simulink model "ASM_Traffic_MultiCore"  (R2026a)
settings: Solver=ode1  StartTime=SIM.tstart.v  StopTime=SIM.tend.v  FixedStep=SIM.StepSize.v
PostLoadFcn:
  | if any(exist('dsrtsu_mdlpostloadfcn', 'file') ~= 0), dsrtsu_mdlpostloadfcn('Execute', bdroot); end
  | try, asm_mdl_postloadfcn(bdroot, 'UpdateModel', 3600); catch, disp(lasterr); end,
InitFcn:
  | , if any(exist('rtifpga_mdlclblib', 'file') ~= 0), rtifpga_mdlclblib('Init', bdroot); end,
  | , if any(exist('dsmpb_private', 'file') ~= 0), dsmpb_private('dsmpb_mdlclblib', 'Init', bdroot); end,
model workspace (MAT data in the model file):
  asmReferencePath = [0 0.01 0.02 0.03 0.04 0.05 0.06 0.07 0.08 0.09 0.1 0.11 ... (350007 elements, 50001x7)]
  roadBounds : Simulink.Parameter (value not decoded)
  safetyAxes : Simulink.Parameter (value not decoded)
undefined symbols (not defined in the file): _to_, a0b2, ASM_BrakeHydraulics_DemoSystems, ASM_VehicleDynamics_DemoSystems, b98103fe8ad365046cd0, BrakeCircuit, controllerConfig, CPT, Crankshaft, DiscIntNeverNeededParam, dsmsi, FinalDriveAssembly, MDL, ModeSignals, mu, Pos_BrakePedal_Maneuver, rad, RefSignals, roadFamilyData, roadFamilyId, s_to_rpm, SIM, SoftECU, Suspension, Tire, Transmission
libraries: ASM_Traffic_lib x135, simulink x98, ASM_Utils_lib x77, ASM_VehicleDynamics_lib x70, ASM_Environment_lib x22, dsmpblib x20, dsmsilib x15, MDLD_Utils_lib x10, ASM_BrakeHydraulics_lib x3, sl_discontinuities x2
(part 42 of 65)

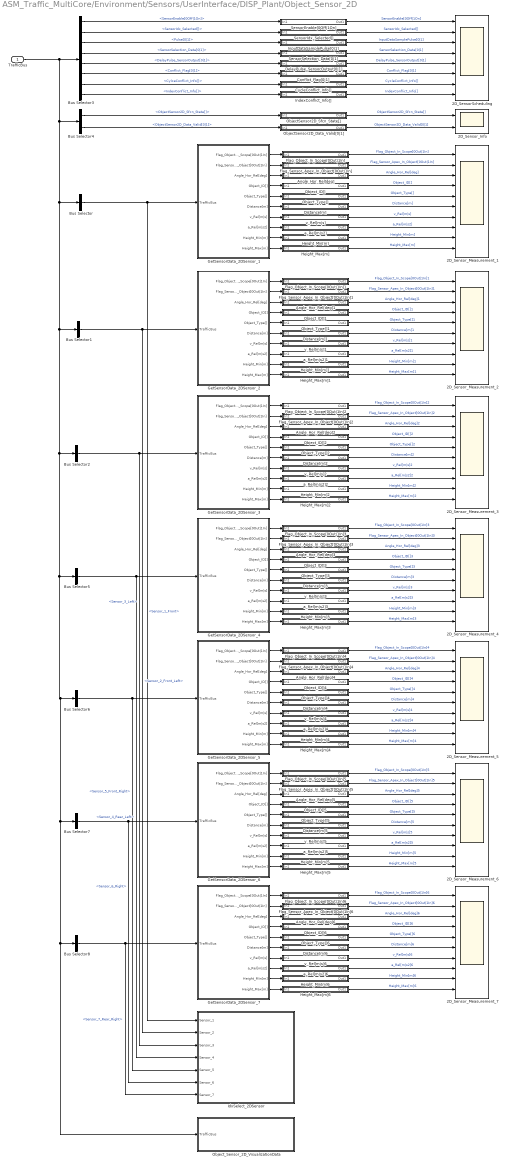
== system ASM_Traffic_MultiCore/Environment/Sensors/UserInterface/DISP_Plant/Object_Sensor_2D ==
  TrafficBus : Inport
  2D_SensorScheduling : Scope  NumInputPorts=8
      settings: TimeSpan=5  ActiveDisplayYMinimum=-0.125  ActiveDisplayYMaximum=1.125  DataLoggingMaxPoints=20000  DataLoggingVariableName=ScopeData36
  2D_Sensor_Info : Scope  NumInputPorts=2
      settings: TimeSpan=5  ActiveDisplayYMinimum=0.75  ActiveDisplayYMaximum=3.25  DataLoggingMaxPoints=20000  DataLoggingVariableName=ScopeData39
  2D_Sensor_Measurement_{1..7} (7 alike) : Scope  NumInputPorts=10
      2D_Sensor_Measurement_1 settings: TimeSpan=5  ActiveDisplayYMinimum=-1  ActiveDisplayYMaximum=1  DataLoggingMaxPoints=20000  DataLoggingDecimation=10  DataLoggingVariableName=ScopeData25
      2D_Sensor_Measurement_2 settings: TimeSpan=5  DataLoggingMaxPoints=20000  DataLoggingDecimation=10  DataLoggingSaveFormat=Array
      2D_Sensor_Measurement_3 settings: TimeSpan=5  DataLoggingMaxPoints=20000  DataLoggingDecimation=10  DataLoggingVariableName=ScopeData2  DataLoggingSaveFormat=Array
      2D_Sensor_Measurement_4 settings: TimeSpan=5  DataLoggingMaxPoints=20000  DataLoggingDecimation=10  DataLoggingVariableName=ScopeData3  DataLoggingSaveFormat=Array
      2D_Sensor_Measurement_5 settings: TimeSpan=5  DataLoggingMaxPoints=20000  DataLoggingDecimation=10  DataLoggingVariableName=ScopeData4  DataLoggingSaveFormat=Array
      2D_Sensor_Measurement_6 settings: TimeSpan=5  DataLoggingMaxPoints=20000  DataLoggingDecimation=10  DataLoggingVariableName=ScopeData5  DataLoggingSaveFormat=Array
      2D_Sensor_Measurement_7 settings: TimeSpan=5  DataLoggingMaxPoints=20000  DataLoggingDecimation=10  DataLoggingVariableName=ScopeData6  DataLoggingSaveFormat=Array
  Angle_Hor_Rel[deg] : Subsystem
      mask Display: disp('')
  Angle_Hor_Rel[deg]1 : Subsystem
      mask Display: disp('')
  Angle_Hor_Rel[deg]2 : Subsystem
      mask Display: disp('')
  Angle_Hor_Rel[deg]3 : Subsystem
      mask Display: disp('')
  Angle_Hor_Rel[deg]4 : Subsystem
      mask Display: disp('')
  Angle_Hor_Rel[deg]5 : Subsystem
      mask Display: disp('')
  Angle_Hor_Rel[deg]6 : Subsystem
      mask Display: disp('')
  Bus Selector : BusSelector  OutputSignals=Object_Sensor_2D.Sensor_1_Front
  Bus Selector1 : BusSelector  OutputSignals=Object_Sensor_2D.Sensor_2_Front_Left
  Bus Selector2 : BusSelector  OutputSignals=Object_Sensor_2D.Sensor_3_Left
  Bus Selector3 : BusSelector  OutputSignals=Object_Sensor_2D.Sensor_Scheduler.SensorEnable[0Off|1On],Object_Sensor_2D.Sensor_Scheduler.SensorIdx_Selected[],Object_Sensor_2D.Sample_Pulse.Pulse[0|1],Object_Sensor_2D.Sensor_Scheduler.SensorSelection_Data[0|1],Object_Sensor_2D.Sensor_Scheduler.DelayPulse_SensorOutput[0|1],Object_Sensor_2D.Sensor_Scheduler.Conflict_Flag[0|1],Object_Sensor_2D.Sensor_Scheduler.CylceConflict_Info[],Object_Sensor_2D.Sensor_Scheduler.IndexConflict_Info[]
  Bus Selector4 : BusSelector  OutputSignals=Object_Sensor_2D.Sensor_1_Front.Info.ObjectSensor2D_Sfcn_State[],Object_Sensor_2D.Sensor_1_Front.Info.ObjectSensor2D_Data_Valid[0|1]
  Bus Selector5 : BusSelector  OutputSignals=Object_Sensor_2D.Sensor_4_Rear_Left
  Bus Selector6 : BusSelector  OutputSignals=Object_Sensor_2D.Sensor_5_Front_Right
  Bus Selector7 : BusSelector  OutputSignals=Object_Sensor_2D.Sensor_6_Right
  Bus Selector8 : BusSelector  OutputSignals=Object_Sensor_2D.Sensor_7_Rear_Right
  Conflict_Flag[0|1] : Subsystem
      mask Display: disp('')
  CycleConflict_Info[] : Subsystem
      mask Display: disp('')
  DelayPulse_SensorOutput[0|1] : Subsystem
      mask Display: disp('')
  Distance[m] : Subsystem
      mask Display: disp('')
  Distance[m]1 : Subsystem
      mask Display: disp('')
  Distance[m]2 : Subsystem
      mask Display: disp('')
  Distance[m]3 : Subsystem
      mask Display: disp('')
  Distance[m]4 : Subsystem
      mask Display: disp('')
  Distance[m]5 : Subsystem
      mask Display: disp('')
  Distance[m]6 : Subsystem
      mask Display: disp('')
  Flag_Object_In_Scope[0Out|1In] : Subsystem
      mask Display: disp('')
  Flag_Object_In_Scope[0Out|1In]1 : Subsystem
      mask Display: disp('')
  Flag_Object_In_Scope[0Out|1In]2 : Subsystem
      mask Display: disp('')
  Flag_Object_In_Scope[0Out|1In]3 : Subsystem
      mask Display: disp('')
  Flag_Object_In_Scope[0Out|1In]4 : Subsystem
      mask Display: disp('')
  Flag_Object_In_Scope[0Out|1In]5 : Subsystem
      mask Display: disp('')
  Flag_Object_In_Scope[0Out|1In]6 : Subsystem
      mask Display: disp('')
  Flag_Sensor_Apex_In_Object[0Out|1In] : Subsystem
      mask Display: disp('')
  Flag_Sensor_Apex_In_Object[0Out|1In]1 : Subsystem
      mask Display: disp('')
  Flag_Sensor_Apex_In_Object[0Out|1In]2 : Subsystem
      mask Display: disp('')
  Flag_Sensor_Apex_In_Object[0Out|1In]3 : Subsystem
      mask Display: disp('')
  Flag_Sensor_Apex_In_Object[0Out|1In]4 : Subsystem
      mask Display: disp('')
  Flag_Sensor_Apex_In_Object[0Out|1In]5 : Subsystem
      mask Display: disp('')
  Flag_Sensor_Apex_In_Object[0Out|1In]6 : Subsystem
      mask Display: disp('')
  GetSensorData_2DSensor_1 : Subsystem
  GetSensorData_2DSensor_2 : Subsystem
  GetSensorData_2DSensor_3 : Subsystem
  GetSensorData_2DSensor_4 : Subsystem
  GetSensorData_2DSensor_5 : Subsystem
  GetSensorData_2DSensor_6 : Subsystem
  GetSensorData_2DSensor_7 : Subsystem
  Height_Max[m] : Subsystem
      mask Display: disp('')
  Height_Max[m]1 : Subsystem
      mask Display: disp('')
  Height_Max[m]2 : Subsystem
      mask Display: disp('')
  Height_Max[m]3 : Subsystem
      mask Display: disp('')
  Height_Max[m]4 : Subsystem
      mask Display: disp('')
  Height_Max[m]5 : Subsystem
      mask Display: disp('')
  Height_Max[m]6 : Subsystem
      mask Display: disp('')
  Height_Min[m] : Subsystem
      mask Display: disp('')
  Height_Min[m]1 : Subsystem
      mask Display: disp('')
  Height_Min[m]2 : Subsystem
      mask Display: disp('')
  Height_Min[m]3 : Subsystem
      mask Display: disp('')
  Height_Min[m]4 : Subsystem
      mask Display: disp('')
  Height_Min[m]5 : Subsystem
      mask Display: disp('')
  Height_Min[m]6 : Subsystem
      mask Display: disp('')
  IdxSelect_2DSensor : Subsystem
  IndexConflict_Info[] : Subsystem
      mask Display: disp('')
  InputDataSamplePulse[0|1] : Subsystem
      mask Display: disp('')
  ObjectSensor2D_Data_Valid[0|1] : Subsystem
      mask Display: disp('')
  ObjectSensor2D_Sfcn_State[] : Subsystem
      mask Display: disp('')
  Object_ID[] : Subsystem
      mask Display: disp('')
  Object_ID[]1 : Subsystem
      mask Display: disp('')
  Object_ID[]2 : Subsystem
      mask Display: disp('')
  Object_ID[]3 : Subsystem
      mask Display: disp('')
  Object_ID[]4 : Subsystem
      mask Display: disp('')
  Object_ID[]5 : Subsystem
      mask Display: disp('')
  Object_ID[]6 : Subsystem
      mask Display: disp('')
  Object_Sensor_2D_VisualizationData : Subsystem
  Object_Type[] : Subsystem
      mask Display: disp('')
  Object_Type[]1 : Subsystem
      mask Display: disp('')
  Object_Type[]2 : Subsystem
      mask Display: disp('')
  Object_Type[]3 : Subsystem
      mask Display: disp('')
  Object_Type[]4 : Subsystem
      mask Display: disp('')
  Object_Type[]5 : Subsystem
      mask Display: disp('')
  Object_Type[]6 : Subsystem
      mask Display: disp('')
  SensorEnable[0Off|1On] : Subsystem
      mask Display: disp('')
  SensorIdx_Selected[] : Subsystem
      mask Display: disp('')
  SensorSelection_Data[0|1] : Subsystem
      mask Display: disp('')
  a_Rel[m|s2] : Subsystem
      mask Display: disp('')
  a_Rel[m|s2]1 : Subsystem
      mask Display: disp('')
  a_Rel[m|s2]2 : Subsystem
      mask Display: disp('')
  a_Rel[m|s2]3 : Subsystem
      mask Display: disp('')
  a_Rel[m|s2]4 : Subsystem
      mask Display: disp('')
  a_Rel[m|s2]5 : Subsystem
      mask Display: disp('')
  a_Rel[m|s2]6 : Subsystem
      mask Display: disp('')
  v_Rel[m|s] : Subsystem
      mask Display: disp('')
  v_Rel[m|s]1 : Subsystem
      mask Display: disp('')
  v_Rel[m|s]2 : Subsystem
      mask Display: disp('')
  v_Rel[m|s]3 : Subsystem
      mask Display: disp('')
  v_Rel[m|s]4 : Subsystem
      mask Display: disp('')
  v_Rel[m|s]5 : Subsystem
      mask Display: disp('')
  v_Rel[m|s]6 : Subsystem
      mask Display: disp('')
  wires:
  GetSensorData_2DSensor_7/1(Flag_Object_In_Scope[0Out|1In]) -> Flag_Object_In_Scope[0Out|1In]6/1(In1)
  GetSensorData_2DSensor_7/2(Flag_Sensor_Apex_In_Object[0Out|1In]) -> Flag_Sensor_Apex_In_Object[0Out|1In]6/1(In1)
  Flag_Object_In_Scope[0Out|1In]6/1(Out1) -> 2D_Sensor_Measurement_7/1  "Flag_Object_In_Scope[0Out|1In]6"
  Flag_Sensor_Apex_In_Object[0Out|1In]6/1(Out1) -> 2D_Sensor_Measurement_7/2  "Flag_Sensor_Apex_In_Object[0Out|1In]6"
  Angle_Hor_Rel[deg]6/1(Out1) -> 2D_Sensor_Measurement_7/3  "Angle_Hor_Rel[deg]6"
  Height_Min[m]6/1(Out1) -> 2D_Sensor_Measurement_7/9  "Height_Min[m]6"
  Height_Max[m]6/1(Out1) -> 2D_Sensor_Measurement_7/10  "Height_Max[m]6"
  a_Rel[m|s2]6/1(Out1) -> 2D_Sensor_Measurement_7/8  "a_Rel[m|s2]6"
  v_Rel[m|s]6/1(Out1) -> 2D_Sensor_Measurement_7/7  "v_Rel[m|s]6"
  Distance[m]6/1(Out1) -> 2D_Sensor_Measurement_7/6  "Distance[m]6"
  Object_Type[]6/1(Out1) -> 2D_Sensor_Measurement_7/5  "Object_Type[]6"
  Object_ID[]6/1(Out1) -> 2D_Sensor_Measurement_7/4  "Object_ID[]6"
  GetSensorData_2DSensor_7/9(Height_Min[m]) -> Height_Min[m]6/1(In1)
  GetSensorData_2DSensor_7/10(Height_Max[m]) -> Height_Max[m]6/1(In1)
  GetSensorData_2DSensor_7/8(a_Rel[m|s2]) -> a_Rel[m|s2]6/1(In1)
  GetSensorData_2DSensor_7/7(v_Rel[m|s]) -> v_Rel[m|s]6/1(In1)
  GetSensorData_2DSensor_7/6(Distance[m]) -> Distance[m]6/1(In1)
  GetSensorData_2DSensor_7/5(Object_Type[]) -> Object_Type[]6/1(In1)
  GetSensorData_2DSensor_7/4(Object_ID[]) -> Object_ID[]6/1(In1)
  GetSensorData_2DSensor_7/3(Angle_Hor_Rel[deg]) -> Angle_Hor_Rel[deg]6/1(In1)
  Bus Selector8/1 -> GetSensorData_2DSensor_7/1(TrafficBus), IdxSelect_2DSensor/7(Sensor_7)  "<Sensor_7_Rear_Right>"
  TrafficBus/1 -> Bus Selector3/1, Bus Selector4/1, Bus Selector/1, Bus Selector1/1, Bus Selector2/1, Bus Selector5/1, Bus Selector6/1, Bus Selector7/1, Bus Selector8/1, Object_Sensor_2D_VisualizationData/1(TrafficBus)
  GetSensorData_2DSensor_6/1(Flag_Object_In_Scope[0Out|1In]) -> Flag_Object_In_Scope[0Out|1In]5/1(In1)
  GetSensorData_2DSensor_6/2(Flag_Sensor_Apex_In_Object[0Out|1In]) -> Flag_Sensor_Apex_In_Object[0Out|1In]5/1(In1)
  Flag_Object_In_Scope[0Out|1In]5/1(Out1) -> 2D_Sensor_Measurement_6/1  "Flag_Object_In_Scope[0Out|1In]5"
  Flag_Sensor_Apex_In_Object[0Out|1In]5/1(Out1) -> 2D_Sensor_Measurement_6/2  "Flag_Sensor_Apex_In_Object[0Out|1In]5"
  Angle_Hor_Rel[deg]5/1(Out1) -> 2D_Sensor_Measurement_6/3  "Angle_Hor_Rel[deg]5"
  Height_Min[m]5/1(Out1) -> 2D_Sensor_Measurement_6/9  "Height_Min[m]5"
  Height_Max[m]5/1(Out1) -> 2D_Sensor_Measurement_6/10  "Height_Max[m]5"
  a_Rel[m|s2]5/1(Out1) -> 2D_Sensor_Measurement_6/8  "a_Rel[m|s2]5"
  v_Rel[m|s]5/1(Out1) -> 2D_Sensor_Measurement_6/7  "v_Rel[m|s]5"
  Distance[m]5/1(Out1) -> 2D_Sensor_Measurement_6/6  "Distance[m]5"
  Object_Type[]5/1(Out1) -> 2D_Sensor_Measurement_6/5  "Object_Type[]5"
  Object_ID[]5/1(Out1) -> 2D_Sensor_Measurement_6/4  "Object_ID[]5"
  GetSensorData_2DSensor_6/9(Height_Min[m]) -> Height_Min[m]5/1(In1)
  GetSensorData_2DSensor_6/10(Height_Max[m]) -> Height_Max[m]5/1(In1)
  GetSensorData_2DSensor_6/8(a_Rel[m|s2]) -> a_Rel[m|s2]5/1(In1)
  GetSensorData_2DSensor_6/7(v_Rel[m|s]) -> v_Rel[m|s]5/1(In1)
  GetSensorData_2DSensor_6/6(Distance[m]) -> Distance[m]5/1(In1)
  GetSensorData_2DSensor_6/5(Object_Type[]) -> Object_Type[]5/1(In1)
  GetSensorData_2DSensor_6/4(Object_ID[]) -> Object_ID[]5/1(In1)
  GetSensorData_2DSensor_6/3(Angle_Hor_Rel[deg]) -> Angle_Hor_Rel[deg]5/1(In1)
  Bus Selector7/1 -> IdxSelect_2DSensor/6(Sensor_6), GetSensorData_2DSensor_6/1(TrafficBus)  "<Sensor_6_Right>"
  GetSensorData_2DSensor_5/1(Flag_Object_In_Scope[0Out|1In]) -> Flag_Object_In_Scope[0Out|1In]4/1(In1)
  GetSensorData_2DSensor_5/2(Flag_Sensor_Apex_In_Object[0Out|1In]) -> Flag_Sensor_Apex_In_Object[0Out|1In]4/1(In1)
  Flag_Object_In_Scope[0Out|1In]4/1(Out1) -> 2D_Sensor_Measurement_5/1  "Flag_Object_In_Scope[0Out|1In]4"
  Flag_Sensor_Apex_In_Object[0Out|1In]4/1(Out1) -> 2D_Sensor_Measurement_5/2  "Flag_Sensor_Apex_In_Object[0Out|1In]4"
  Angle_Hor_Rel[deg]4/1(Out1) -> 2D_Sensor_Measurement_5/3  "Angle_Hor_Rel[deg]4"
  Height_Min[m]4/1(Out1) -> 2D_Sensor_Measurement_5/9  "Height_Min[m]4"
  Height_Max[m]4/1(Out1) -> 2D_Sensor_Measurement_5/10  "Height_Max[m]4"
  a_Rel[m|s2]4/1(Out1) -> 2D_Sensor_Measurement_5/8  "a_Rel[m|s2]4"
  v_Rel[m|s]4/1(Out1) -> 2D_Sensor_Measurement_5/7  "v_Rel[m|s]4"
  Distance[m]4/1(Out1) -> 2D_Sensor_Measurement_5/6  "Distance[m]4"
  Object_Type[]4/1(Out1) -> 2D_Sensor_Measurement_5/5  "Object_Type[]4"
  Object_ID[]4/1(Out1) -> 2D_Sensor_Measurement_5/4  "Object_ID[]4"
  GetSensorData_2DSensor_5/9(Height_Min[m]) -> Height_Min[m]4/1(In1)
  GetSensorData_2DSensor_5/10(Height_Max[m]) -> Height_Max[m]4/1(In1)
  GetSensorData_2DSensor_5/8(a_Rel[m|s2]) -> a_Rel[m|s2]4/1(In1)
  GetSensorData_2DSensor_5/7(v_Rel[m|s]) -> v_Rel[m|s]4/1(In1)
  GetSensorData_2DSensor_5/6(Distance[m]) -> Distance[m]4/1(In1)
  GetSensorData_2DSensor_5/5(Object_Type[]) -> Object_Type[]4/1(In1)
  GetSensorData_2DSensor_5/4(Object_ID[]) -> Object_ID[]4/1(In1)
  GetSensorData_2DSensor_5/3(Angle_Hor_Rel[deg]) -> Angle_Hor_Rel[deg]4/1(In1)
  Bus Selector6/1 -> IdxSelect_2DSensor/5(Sensor_5), GetSensorData_2DSensor_5/1(TrafficBus)  "<Sensor_5_Front_Right>"
  GetSensorData_2DSensor_4/1(Flag_Object_In_Scope[0Out|1In]) -> Flag_Object_In_Scope[0Out|1In]3/1(In1)
  GetSensorData_2DSensor_4/2(Flag_Sensor_Apex_In_Object[0Out|1In]) -> Flag_Sensor_Apex_In_Object[0Out|1In]3/1(In1)
  Flag_Object_In_Scope[0Out|1In]3/1(Out1) -> 2D_Sensor_Measurement_4/1  "Flag_Object_In_Scope[0Out|1In]3"
  Flag_Sensor_Apex_In_Object[0Out|1In]3/1(Out1) -> 2D_Sensor_Measurement_4/2  "Flag_Sensor_Apex_In_Object[0Out|1In]3"
  Angle_Hor_Rel[deg]3/1(Out1) -> 2D_Sensor_Measurement_4/3  "Angle_Hor_Rel[deg]3"
  Height_Min[m]3/1(Out1) -> 2D_Sensor_Measurement_4/9  "Height_Min[m]3"
  Height_Max[m]3/1(Out1) -> 2D_Sensor_Measurement_4/10  "Height_Max[m]3"
  a_Rel[m|s2]3/1(Out1) -> 2D_Sensor_Measurement_4/8  "a_Rel[m|s2]3"
  v_Rel[m|s]3/1(Out1) -> 2D_Sensor_Measurement_4/7  "v_Rel[m|s]3"
  Distance[m]3/1(Out1) -> 2D_Sensor_Measurement_4/6  "Distance[m]3"
  Object_Type[]3/1(Out1) -> 2D_Sensor_Measurement_4/5  "Object_Type[]3"
  Object_ID[]3/1(Out1) -> 2D_Sensor_Measurement_4/4  "Object_ID[]3"
  GetSensorData_2DSensor_4/9(Height_Min[m]) -> Height_Min[m]3/1(In1)
  GetSensorData_2DSensor_4/10(Height_Max[m]) -> Height_Max[m]3/1(In1)
  GetSensorData_2DSensor_4/8(a_Rel[m|s2]) -> a_Rel[m|s2]3/1(In1)
  GetSensorData_2DSensor_4/7(v_Rel[m|s]) -> v_Rel[m|s]3/1(In1)
  GetSensorData_2DSensor_4/6(Distance[m]) -> Distance[m]3/1(In1)
  GetSensorData_2DSensor_4/5(Object_Type[]) -> Object_Type[]3/1(In1)
  GetSensorData_2DSensor_4/4(Object_ID[]) -> Object_ID[]3/1(In1)
  GetSensorData_2DSensor_4/3(Angle_Hor_Rel[deg]) -> Angle_Hor_Rel[deg]3/1(In1)
  Bus Selector5/1 -> IdxSelect_2DSensor/4(Sensor_4), GetSensorData_2DSensor_4/1(TrafficBus)  "<Sensor_4_Rear_Left>"
  GetSensorData_2DSensor_3/1(Flag_Object_In_Scope[0Out|1In]) -> Flag_Object_In_Scope[0Out|1In]2/1(In1)
  GetSensorData_2DSensor_3/2(Flag_Sensor_Apex_In_Object[0Out|1In]) -> Flag_Sensor_Apex_In_Object[0Out|1In]2/1(In1)
  Flag_Object_In_Scope[0Out|1In]2/1(Out1) -> 2D_Sensor_Measurement_3/1  "Flag_Object_In_Scope[0Out|1In]2"
  Flag_Sensor_Apex_In_Object[0Out|1In]2/1(Out1) -> 2D_Sensor_Measurement_3/2  "Flag_Sensor_Apex_In_Object[0Out|1In]2"
  Angle_Hor_Rel[deg]2/1(Out1) -> 2D_Sensor_Measurement_3/3  "Angle_Hor_Rel[deg]2"
  Height_Min[m]2/1(Out1) -> 2D_Sensor_Measurement_3/9  "Height_Min[m]2"
  Height_Max[m]2/1(Out1) -> 2D_Sensor_Measurement_3/10  "Height_Max[m]2"
  a_Rel[m|s2]2/1(Out1) -> 2D_Sensor_Measurement_3/8  "a_Rel[m|s2]2"
  v_Rel[m|s]2/1(Out1) -> 2D_Sensor_Measurement_3/7  "v_Rel[m|s]2"
  Distance[m]2/1(Out1) -> 2D_Sensor_Measurement_3/6  "Distance[m]2"
  Object_Type[]2/1(Out1) -> 2D_Sensor_Measurement_3/5  "Object_Type[]2"
  Object_ID[]2/1(Out1) -> 2D_Sensor_Measurement_3/4  "Object_ID[]2"
  GetSensorData_2DSensor_3/9(Height_Min[m]) -> Height_Min[m]2/1(In1)
  GetSensorData_2DSensor_3/10(Height_Max[m]) -> Height_Max[m]2/1(In1)
  GetSensorData_2DSensor_3/8(a_Rel[m|s2]) -> a_Rel[m|s2]2/1(In1)
  GetSensorData_2DSensor_3/7(v_Rel[m|s]) -> v_Rel[m|s]2/1(In1)
  GetSensorData_2DSensor_3/6(Distance[m]) -> Distance[m]2/1(In1)
  GetSensorData_2DSensor_3/5(Object_Type[]) -> Object_Type[]2/1(In1)
  GetSensorData_2DSensor_3/4(Object_ID[]) -> Object_ID[]2/1(In1)
  GetSensorData_2DSensor_3/3(Angle_Hor_Rel[deg]) -> Angle_Hor_Rel[deg]2/1(In1)
  Bus Selector2/1 -> IdxSelect_2DSensor/3(Sensor_3), GetSensorData_2DSensor_3/1(TrafficBus)  "<Sensor_3_Left>"
  GetSensorData_2DSensor_2/1(Flag_Object_In_Scope[0Out|1In]) -> Flag_Object_In_Scope[0Out|1In]1/1(In1)
  GetSensorData_2DSensor_2/2(Flag_Sensor_Apex_In_Object[0Out|1In]) -> Flag_Sensor_Apex_In_Object[0Out|1In]1/1(In1)
  Flag_Object_In_Scope[0Out|1In]1/1(Out1) -> 2D_Sensor_Measurement_2/1  "Flag_Object_In_Scope[0Out|1In]1"
  Flag_Sensor_Apex_In_Object[0Out|1In]1/1(Out1) -> 2D_Sensor_Measurement_2/2  "Flag_Sensor_Apex_In_Object[0Out|1In]1"
  Angle_Hor_Rel[deg]1/1(Out1) -> 2D_Sensor_Measurement_2/3  "Angle_Hor_Rel[deg]1"
  Height_Min[m]1/1(Out1) -> 2D_Sensor_Measurement_2/9  "Height_Min[m]1"
  Height_Max[m]1/1(Out1) -> 2D_Sensor_Measurement_2/10  "Height_Max[m]1"
  a_Rel[m|s2]1/1(Out1) -> 2D_Sensor_Measurement_2/8  "a_Rel[m|s2]1"
  v_Rel[m|s]1/1(Out1) -> 2D_Sensor_Measurement_2/7  "v_Rel[m|s]1"
  Distance[m]1/1(Out1) -> 2D_Sensor_Measurement_2/6  "Distance[m]1"
  Object_Type[]1/1(Out1) -> 2D_Sensor_Measurement_2/5  "Object_Type[]1"
  Object_ID[]1/1(Out1) -> 2D_Sensor_Measurement_2/4  "Object_ID[]1"
  GetSensorData_2DSensor_2/9(Height_Min[m]) -> Height_Min[m]1/1(In1)
  GetSensorData_2DSensor_2/10(Height_Max[m]) -> Height_Max[m]1/1(In1)
  GetSensorData_2DSensor_2/8(a_Rel[m|s2]) -> a_Rel[m|s2]1/1(In1)
  GetSensorData_2DSensor_2/7(v_Rel[m|s]) -> v_Rel[m|s]1/1(In1)
  GetSensorData_2DSensor_2/6(Distance[m]) -> Distance[m]1/1(In1)
  GetSensorData_2DSensor_2/5(Object_Type[]) -> Object_Type[]1/1(In1)
  GetSensorData_2DSensor_2/4(Object_ID[]) -> Object_ID[]1/1(In1)
  GetSensorData_2DSensor_2/3(Angle_Hor_Rel[deg]) -> Angle_Hor_Rel[deg]1/1(In1)
  GetSensorData_2DSensor_1/1(Flag_Object_In_Scope[0Out|1In]) -> Flag_Object_In_Scope[0Out|1In]/1(In1)
  GetSensorData_2DSensor_1/2(Flag_Sensor_Apex_In_Object[0Out|1In]) -> Flag_Sensor_Apex_In_Object[0Out|1In]/1(In1)
  Flag_Object_In_Scope[0Out|1In]/1(Out1) -> 2D_Sensor_Measurement_1/1  "Flag_Object_In_Scope[0Out|1In]"
  Flag_Sensor_Apex_In_Object[0Out|1In]/1(Out1) -> 2D_Sensor_Measurement_1/2  "Flag_Sensor_Apex_In_Object[0Out|1In]"
  Bus Selector1/1 -> IdxSelect_2DSensor/2(Sensor_2), GetSensorData_2DSensor_2/1(TrafficBus)  "<Sensor_2_Front_Left>"
  ObjectSensor2D_Data_Valid[0|1]/1(Out1) -> 2D_Sensor_Info/2  "ObjectSensor2D_Data_Valid[0|1]"
  ObjectSensor2D_Sfcn_State[]/1(Out1) -> 2D_Sensor_Info/1  "ObjectSensor2D_Sfcn_State[]"
  Bus Selector4/2 -> ObjectSensor2D_Data_Valid[0|1]/1(In1)  "<ObjectSensor2D_Data_Valid[0|1]>"
  Bus Selector4/1 -> ObjectSensor2D_Sfcn_State[]/1(In1)  "<ObjectSensor2D_Sfcn_State[]>"
  Angle_Hor_Rel[deg]/1(Out1) -> 2D_Sensor_Measurement_1/3  "Angle_Hor_Rel[deg]"
  SensorIdx_Selected[]/1(Out1) -> 2D_SensorScheduling/2  "SensorIdx_Selected[]"
  IndexConflict_Info[]/1(Out1) -> 2D_SensorScheduling/8  "IndexConflict_Info[]"
  Bus Selector3/8 -> IndexConflict_Info[]/1(In1)  "<IndexConflict_Info[]>"
  Bus Selector3/7 -> CycleConflict_Info[]/1(In1)  "<CylceConflict_Info[]>"
  Bus Selector3/2 -> SensorIdx_Selected[]/1(In1)  "<SensorIdx_Selected[]>"
  CycleConflict_Info[]/1(Out1) -> 2D_SensorScheduling/7  "CycleConflict_Info[]"
  Conflict_Flag[0|1]/1(Out1) -> 2D_SensorScheduling/6  "Conflict_Flag[0|1]"
  DelayPulse_SensorOutput[0|1]/1(Out1) -> 2D_SensorScheduling/5  "DelayPulse_SensorOutput[0|1]"
  SensorSelection_Data[0|1]/1(Out1) -> 2D_SensorScheduling/4  "SensorSelection_Data[0|1]"
  Bus Selector3/3 -> InputDataSamplePulse[0|1]/1(In1)  "<Pulse[0|1]>"
  Bus Selector3/1 -> SensorEnable[0Off|1On]/1(In1)  "<SensorEnable[0Off|1On]>"
  InputDataSamplePulse[0|1]/1(Out1) -> 2D_SensorScheduling/3  "InputDataSamplePulse[0|1]"
  SensorEnable[0Off|1On]/1(Out1) -> 2D_SensorScheduling/1  "SensorEnable[0Off|1On]"
  Bus Selector3/6 -> Conflict_Flag[0|1]/1(In1)  "<Conflict_Flag[0|1]>"
  Bus Selector3/5 -> DelayPulse_SensorOutput[0|1]/1(In1)  "<DelayPulse_SensorOutput[0|1]>"
  Bus Selector3/4 -> SensorSelection_Data[0|1]/1(In1)  "<SensorSelection_Data[0|1]>"
  Bus Selector/1 -> IdxSelect_2DSensor/1(Sensor_1), GetSensorData_2DSensor_1/1(TrafficBus)  "<Sensor_1_Front>"
  Height_Min[m]/1(Out1) -> 2D_Sensor_Measurement_1/9  "Height_Min[m]"
  Height_Max[m]/1(Out1) -> 2D_Sensor_Measurement_1/10  "Height_Max[m]"
  a_Rel[m|s2]/1(Out1) -> 2D_Sensor_Measurement_1/8  "a_Rel[m|s2]"
  v_Rel[m|s]/1(Out1) -> 2D_Sensor_Measurement_1/7  "v_Rel[m|s]"
  Distance[m]/1(Out1) -> 2D_Sensor_Measurement_1/6  "Distance[m]"
  Object_Type[]/1(Out1) -> 2D_Sensor_Measurement_1/5  "Object_Type[]"
  Object_ID[]/1(Out1) -> 2D_Sensor_Measurement_1/4  "Object_ID[]"
  GetSensorData_2DSensor_1/9(Height_Min[m]) -> Height_Min[m]/1(In1)
  GetSensorData_2DSensor_1/10(Height_Max[m]) -> Height_Max[m]/1(In1)
  GetSensorData_2DSensor_1/8(a_Rel[m|s2]) -> a_Rel[m|s2]/1(In1)
  GetSensorData_2DSensor_1/7(v_Rel[m|s]) -> v_Rel[m|s]/1(In1)
  GetSensorData_2DSensor_1/6(Distance[m]) -> Distance[m]/1(In1)
  GetSensorData_2DSensor_1/5(Object_Type[]) -> Object_Type[]/1(In1)
  GetSensorData_2DSensor_1/4(Object_ID[]) -> Object_ID[]/1(In1)
  GetSensorData_2DSensor_1/3(Angle_Hor_Rel[deg]) -> Angle_Hor_Rel[deg]/1(In1)

== system ASM_Traffic_MultiCore/Environment/Sensors/UserInterface/DISP_Plant/Object_Sensor_3D ==
  TrafficBus : Inport
  3D_Sensor_Info_1 : Scope  NumInputPorts=5
      settings: TimeSpan=5  ActiveDisplayYMinimum=-0.125  ActiveDisplayYMaximum=1.125  DataLoggingMaxPoints=20000  DataLoggingDecimation=10  DataLoggingVariableName=ScopeData24
  3D_Sensor_Info_2 : Scope  NumInputPorts=5
      settings: TimeSpan=5  ActiveDisplayYMinimum=-1  ActiveDisplayYMaximum=1  DataLoggingMaxPoints=20000  DataLoggingDecimation=10  DataLoggingVariableName=ScopeData26
  3D_Sensor_Info_3 : Scope  NumInputPorts=5
      settings: TimeSpan=5  ActiveDisplayYMinimum=0.95  ActiveDisplayYMaximum=1.05  DataLoggingMaxPoints=20000  DataLoggingDecimation=10  DataLoggingVariableName=ScopeData28
  3D_Sensor_Measurement_1 : Scope  NumInputPorts=7
      settings: TimeSpan=5  ActiveDisplayYMinimum=-16.80573  ActiveDisplayYMaximum=141.25157  DataLoggingMaxPoints=20000  DataLoggingDecimation=10  DataLoggingVariableName=ScopeData25
  3D_Sensor_Measurement_2 : Scope  NumInputPorts=7
      settings: TimeSpan=5  ActiveDisplayYMinimum=-9.24144  ActiveDisplayYMaximum=73.17296  DataLoggingMaxPoints=20000  DataLoggingDecimation=10  DataLoggingVariableName=ScopeData27
  3D_Sensor_Measurement_3 : Scope  NumInputPorts=7
      settings: TimeSpan=5  ActiveDisplayYMinimum=-1.1  ActiveDisplayYMaximum=-0.9  DataLoggingMaxPoints=20000  DataLoggingDecimation=10  DataLoggingVariableName=ScopeData29
  Angle_Hor_Object[deg] : Subsystem
      mask Display: disp('')
  Angle_Hor_Object[deg]1 : Subsystem
      mask Display: disp('')
  Angle_Hor_Object[deg]2 : Subsystem
      mask Display: disp('')
  Angle_Ver_Object[deg] : Subsystem
      mask Display: disp('')
  Angle_Ver_Object[deg]1 : Subsystem
      mask Display: disp('')
  Angle_Ver_Object[deg]2 : Subsystem
      mask Display: disp('')
  Bus Selector : BusSelector  OutputSignals=Object_Sensor_3D.Sensor_1_Front_Long
  Bus Selector1 : BusSelector  OutputSignals=Object_Sensor_3D.Sensor_2_Front_Mid
  Bus Selector2 : BusSelector  OutputSignals=Object_Sensor_3D.Sensor_3_Rear
  Bus Selector3 : BusSelector  OutputSignals=Object_Sensor_3D.Sensor_Scheduler.SensorEnable[0Off|1On],Object_Sensor_3D.Sensor_Scheduler.SensorIdx_Selected[],Object_Sensor_3D.Sample_Pulse.Pulse[0|1],Object_Sensor_3D.Sensor_Scheduler.SensorSelection_Data[0|1],Object_Sensor_3D.Sensor_Scheduler.DelayPulse_SensorOutput[0|1],Object_Sensor_3D.Sensor_Scheduler.Conflict_Flag[0|1],Object_Sensor_3D.Sensor_Scheduler.CylceConflict_Info[],Object_Sensor_3D.Sensor_Scheduler.IndexConflict_Info[]
  Conflict_Flag[0|1] : Subsystem
      mask Display: disp('')
  CycleConflict_Info[] : Subsystem
      mask Display: disp('')
  DelayPulse_SensorOutput[0|1] : Subsystem
      mask Display: disp('')
  Dist_Object[m] : Subsystem
      mask Display: disp('')
  Dist_Object[m]1 : Subsystem
      mask Display: disp('')
  Dist_Object[m]2 : Subsystem
      mask Display: disp('')
  Flag_NearestPnt_Occluded[-1|0|1] : Subsystem
      mask Display: disp('')
  Flag_NearestPnt_Occluded[-1|0|1]1 : Subsystem
      mask Display: disp('')
  Flag_NearestPnt_Occluded[-1|0|1]2 : Subsystem
      mask Display: disp('')
  Flag_Object_In_Scope[0Out|1In] : Subsystem
      mask Display: disp('')
  Flag_Object_In_Scope[0Out|1In]1 : Subsystem
      mask Display: disp('')
  Flag_Object_In_Scope[0Out|1In]2 : Subsystem
      mask Display: disp('')
  Flag_Sensor_Apex_In_Object[0Out|1In] : Subsystem
      mask Display: disp('')
  Flag_Sensor_Apex_In_Object[0Out|1In]1 : Subsystem
      mask Display: disp('')
  Flag_Sensor_Apex_In_Object[0Out|1In]2 : Subsystem
      mask Display: disp('')
  GetSensorData_3DSensor_1 : Subsystem
  GetSensorData_3DSensor_2 : Subsystem
  GetSensorData_3DSensor_3 : Subsystem
  IdxSelect_3DSensor : Subsystem
  IndexConflict_Info[] : Subsystem
      mask Display: disp('')
  InputDataSamplePulse[0|1] : Subsystem
      mask Display: disp('')
  Object_ID[] : Subsystem
      mask Display: disp('')
  Object_ID[]1 : Subsystem
      mask Display: disp('')
  Object_ID[]2 : Subsystem
      mask Display: disp('')
  Object_Info[-1None|1Fellow|2Static] : Subsystem
      mask Display: disp('')
  Object_Info[-1None|1Fellow|2Static]1 : Subsystem
      mask Display: disp('')
  Object_Info[-1None|1Fellow|2Static]2 : Subsystem
      mask Display: disp('')
  Object_Sensor_3D_VisualizationData : Subsystem
  Object_Type[] : Subsystem
      mask Display: disp('')
  Object_Type[]1 : Subsystem
      mask Display: disp('')
  Object_Type[]2 : Subsystem
      mask Display: disp('')
  Occlusion_Ratio_Object[-1|0_1] : Subsystem
      mask Display: disp('')
  Occlusion_Ratio_Object[-1|0_1]1 : Subsystem
      mask Display: disp('')
  Occlusion_Ratio_Object[-1|0_1]2 : Subsystem
      mask Display: disp('')
  SensorEnable[0Off|1On] : Subsystem
      mask Display: disp('')
  SensorIdx_Selected[] : Subsystem
      mask Display: disp('')
  SensorScheduling : Scope  NumInputPorts=8
      settings: TimeSpan=5  ActiveDisplayYMinimum=-5  ActiveDisplayYMaximum=5  DataLoggingMaxPoints=20000  DataLoggingVariableName=ScopeData36
  SensorSelection_Data[0|1] : Subsystem
      mask Display: disp('')
  a_Rel_Object[m|s2] : Subsystem
      mask Display: disp('')
  a_Rel_Object[m|s2]1 : Subsystem
      mask Display: disp('')
  a_Rel_Object[m|s2]2 : Subsystem
      mask Display: disp('')
  v_Rel_Object[m|s] : Subsystem
      mask Display: disp('')
  v_Rel_Object[m|s]1 : Subsystem
      mask Display: disp('')
  v_Rel_Object[m|s]2 : Subsystem
      mask Display: disp('')
  wires:
  Flag_NearestPnt_Occluded[-1|0|1]2/1(Out1) -> 3D_Sensor_Measurement_3/7  "Flag_NearestPnt_Occluded[-1|0|1]2"
  GetSensorData_3DSensor_3/12(Flag_NearestPnt_Occluded[-1|0|1]) -> Flag_NearestPnt_Occluded[-1|0|1]2/1(In1)
  Occlusion_Ratio_Object[-1|0_1]2/1(Out1) -> 3D_Sensor_Measurement_3/6  "Occlusion_Ratio_Object[-1|0_1]2"
  GetSensorData_3DSensor_3/11(Occlusion_Ratio_Object[-1|0_1]) -> Occlusion_Ratio_Object[-1|0_1]2/1(In1)
  GetSensorData_3DSensor_2/11(Occlusion_Ratio_Object[-1|0_1]) -> Occlusion_Ratio_Object[-1|0_1]1/1(In1)
  Occlusion_Ratio_Object[-1|0_1]1/1(Out1) -> 3D_Sensor_Measurement_2/6  "Occlusion_Ratio_Object[-1|0_1]1"
  GetSensorData_3DSensor_2/12(Flag_NearestPnt_Occluded[-1|0|1]) -> Flag_NearestPnt_Occluded[-1|0|1]1/1(In1)
  Flag_NearestPnt_Occluded[-1|0|1]1/1(Out1) -> 3D_Sensor_Measurement_2/7  "Flag_NearestPnt_Occluded[-1|0|1]1"
  GetSensorData_3DSensor_2/10(Angle_Ver_Object[deg]) -> Angle_Ver_Object[deg]1/1(In1)
  GetSensorData_3DSensor_2/9(Angle_Hor_Object[deg]) -> Angle_Hor_Object[deg]1/1(In1)
  GetSensorData_3DSensor_2/8(a_Rel_Object[m|s2]) -> a_Rel_Object[m|s2]1/1(In1)
  GetSensorData_3DSensor_2/7(v_Rel_Object[m|s]) -> v_Rel_Object[m|s]1/1(In1)
  GetSensorData_3DSensor_2/6(Dist_Object[m]) -> Dist_Object[m]1/1(In1)
  GetSensorData_3DSensor_2/5(Object_Type[]) -> Object_Type[]1/1(In1)
  GetSensorData_3DSensor_2/4(Object_ID[]) -> Object_ID[]1/1(In1)
  GetSensorData_3DSensor_2/3(Object_Info[-1None|1Fellow|2Static]) -> Object_Info[-1None|1Fellow|2Static]1/1(In1)
  GetSensorData_3DSensor_2/2(Flag_Sensor_Apex_In_Object[0Out|1In]) -> Flag_Sensor_Apex_In_Object[0Out|1In]1/1(In1)
  GetSensorData_3DSensor_2/1(Flag_Object_In_Scope[0Out|1In]) -> Flag_Object_In_Scope[0Out|1In]1/1(In1)
  Flag_NearestPnt_Occluded[-1|0|1]/1(Out1) -> 3D_Sensor_Measurement_1/7  "Flag_NearestPnt_Occluded[-1|0|1]"
  Occlusion_Ratio_Object[-1|0_1]/1(Out1) -> 3D_Sensor_Measurement_1/6  "Occlusion_Ratio_Object[-1|0_1]"
  GetSensorData_3DSensor_1/12(Flag_NearestPnt_Occluded[-1|0|1]) -> Flag_NearestPnt_Occluded[-1|0|1]/1(In1)
  GetSensorData_3DSensor_1/11(Occlusion_Ratio_Object[-1|0_1]) -> Occlusion_Ratio_Object[-1|0_1]/1(In1)
  TrafficBus/1 -> Bus Selector1/1, Bus Selector2/1, Object_Sensor_3D_VisualizationData/1(TrafficBus), Bus Selector/1, Bus Selector3/1
  GetSensorData_3DSensor_1/1(Flag_Object_In_Scope[0Out|1In]) -> Flag_Object_In_Scope[0Out|1In]/1(In1)
  GetSensorData_3DSensor_1/2(Flag_Sensor_Apex_In_Object[0Out|1In]) -> Flag_Sensor_Apex_In_Object[0Out|1In]/1(In1)
  GetSensorData_3DSensor_1/3(Object_Info[-1None|1Fellow|2Static]) -> Object_Info[-1None|1Fellow|2Static]/1(In1)
  GetSensorData_3DSensor_1/4(Object_ID[]) -> Object_ID[]/1(In1)
  GetSensorData_3DSensor_1/5(Object_Type[]) -> Object_Type[]/1(In1)
  GetSensorData_3DSensor_1/6(Dist_Object[m]) -> Dist_Object[m]/1(In1)
  GetSensorData_3DSensor_1/7(v_Rel_Object[m|s]) -> v_Rel_Object[m|s]/1(In1)
  GetSensorData_3DSensor_1/8(a_Rel_Object[m|s2]) -> a_Rel_Object[m|s2]/1(In1)
  GetSensorData_3DSensor_1/9(Angle_Hor_Object[deg]) -> Angle_Hor_Object[deg]/1(In1)
  GetSensorData_3DSensor_1/10(Angle_Ver_Object[deg]) -> Angle_Ver_Object[deg]/1(In1)
  Flag_Object_In_Scope[0Out|1In]/1(Out1) -> 3D_Sensor_Info_1/1  "Flag_Object_In_Scope[0Out|1In]"
  Flag_Sensor_Apex_In_Object[0Out|1In]/1(Out1) -> 3D_Sensor_Info_1/2  "Flag_Sensor_Apex_In_Object[0Out|1In]"
  Object_Info[-1None|1Fellow|2Static]/1(Out1) -> 3D_Sensor_Info_1/3  "Object_Info[-1None|1Fellow|2Static]"
  Object_ID[]/1(Out1) -> 3D_Sensor_Info_1/4  "Object_ID[]"
  Object_Type[]/1(Out1) -> 3D_Sensor_Info_1/5  "Object_Type[]"
  Dist_Object[m]/1(Out1) -> 3D_Sensor_Measurement_1/1  "Dist_Object[m]"
  v_Rel_Object[m|s]/1(Out1) -> 3D_Sensor_Measurement_1/2  "v_Rel_Object[m|s]"
  a_Rel_Object[m|s2]/1(Out1) -> 3D_Sensor_Measurement_1/3  "a_Rel_Object[m|s2]"
  Angle_Hor_Object[deg]/1(Out1) -> 3D_Sensor_Measurement_1/4  "Angle_Hor_Object[deg]"
  Angle_Ver_Object[deg]/1(Out1) -> 3D_Sensor_Measurement_1/5  "Angle_Ver_Object[deg]"
  Flag_Object_In_Scope[0Out|1In]1/1(Out1) -> 3D_Sensor_Info_2/1  "Flag_Object_In_Scope[0Out|1In]1"
  Flag_Sensor_Apex_In_Object[0Out|1In]1/1(Out1) -> 3D_Sensor_Info_2/2  "Flag_Sensor_Apex_In_Object[0Out|1In]1"
  Object_Info[-1None|1Fellow|2Static]1/1(Out1) -> 3D_Sensor_Info_2/3  "Object_Info[-1None|1Fellow|2Static]1"
  Object_ID[]1/1(Out1) -> 3D_Sensor_Info_2/4  "Object_ID[]1"
  Object_Type[]1/1(Out1) -> 3D_Sensor_Info_2/5  "Object_Type[]1"
  Dist_Object[m]1/1(Out1) -> 3D_Sensor_Measurement_2/1  "Dist_Object[m]1"
  v_Rel_Object[m|s]1/1(Out1) -> 3D_Sensor_Measurement_2/2  "v_Rel_Object[m|s]1"
  a_Rel_Object[m|s2]1/1(Out1) -> 3D_Sensor_Measurement_2/3  "a_Rel_Object[m|s2]1"
  Angle_Hor_Object[deg]1/1(Out1) -> 3D_Sensor_Measurement_2/4  "Angle_Hor_Object[deg]1"
  Angle_Ver_Object[deg]1/1(Out1) -> 3D_Sensor_Measurement_2/5  "Angle_Ver_Object[deg]1"
  Flag_Object_In_Scope[0Out|1In]2/1(Out1) -> 3D_Sensor_Info_3/1  "Flag_Object_In_Scope[0Out|1In]2"
  Flag_Sensor_Apex_In_Object[0Out|1In]2/1(Out1) -> 3D_Sensor_Info_3/2  "Flag_Sensor_Apex_In_Object[0Out|1In]2"
  Object_Info[-1None|1Fellow|2Static]2/1(Out1) -> 3D_Sensor_Info_3/3  "Object_Info[-1None|1Fellow|2Static]2"
  Object_ID[]2/1(Out1) -> 3D_Sensor_Info_3/4  "Object_ID[]2"
  Object_Type[]2/1(Out1) -> 3D_Sensor_Info_3/5  "Object_Type[]2"
  Dist_Object[m]2/1(Out1) -> 3D_Sensor_Measurement_3/1  "Dist_Object[m]2"
  v_Rel_Object[m|s]2/1(Out1) -> 3D_Sensor_Measurement_3/2  "v_Rel_Object[m|s]2"
  a_Rel_Object[m|s2]2/1(Out1) -> 3D_Sensor_Measurement_3/3  "a_Rel_Object[m|s2]2"
  Angle_Hor_Object[deg]2/1(Out1) -> 3D_Sensor_Measurement_3/4  "Angle_Hor_Object[deg]2"
  Angle_Ver_Object[deg]2/1(Out1) -> 3D_Sensor_Measurement_3/5  "Angle_Ver_Object[deg]2"
  GetSensorData_3DSensor_3/1(Flag_Object_In_Scope[0Out|1In]) -> Flag_Object_In_Scope[0Out|1In]2/1(In1)
  GetSensorData_3DSensor_3/2(Flag_Sensor_Apex_In_Object[0Out|1In]) -> Flag_Sensor_Apex_In_Object[0Out|1In]2/1(In1)
  GetSensorData_3DSensor_3/3(Object_Info[-1None|1Fellow|2Static]) -> Object_Info[-1None|1Fellow|2Static]2/1(In1)
  GetSensorData_3DSensor_3/4(Object_ID[]) -> Object_ID[]2/1(In1)
  GetSensorData_3DSensor_3/5(Object_Type[]) -> Object_Type[]2/1(In1)
  GetSensorData_3DSensor_3/6(Dist_Object[m]) -> Dist_Object[m]2/1(In1)
  GetSensorData_3DSensor_3/7(v_Rel_Object[m|s]) -> v_Rel_Object[m|s]2/1(In1)
  GetSensorData_3DSensor_3/8(a_Rel_Object[m|s2]) -> a_Rel_Object[m|s2]2/1(In1)
  GetSensorData_3DSensor_3/9(Angle_Hor_Object[deg]) -> Angle_Hor_Object[deg]2/1(In1)
  GetSensorData_3DSensor_3/10(Angle_Ver_Object[deg]) -> Angle_Ver_Object[deg]2/1(In1)
  Bus Selector/1 -> IdxSelect_3DSensor/1(Sensor_1), GetSensorData_3DSensor_1/1(TrafficBus)  "<Sensor_1_Front_Long>"
  Bus Selector1/1 -> IdxSelect_3DSensor/2(Sensor_2), GetSensorData_3DSensor_2/1(TrafficBus)  "<Sensor_2_Front_Mid>"
  Bus Selector2/1 -> IdxSelect_3DSensor/3(Sensor_3), GetSensorData_3DSensor_3/1(TrafficBus)  "<Sensor_3_Rear>"
  Bus Selector3/4 -> SensorSelection_Data[0|1]/1(In1)  "<SensorSelection_Data[0|1]>"
  Bus Selector3/5 -> DelayPulse_SensorOutput[0|1]/1(In1)  "<DelayPulse_SensorOutput[0|1]>"
  Bus Selector3/6 -> Conflict_Flag[0|1]/1(In1)  "<Conflict_Flag[0|1]>"
  SensorEnable[0Off|1On]/1(Out1) -> SensorScheduling/1  "SensorEnable[0Off|1On]"
  InputDataSamplePulse[0|1]/1(Out1) -> SensorScheduling/3  "InputDataSamplePulse[0|1]"
  Bus Selector3/1 -> SensorEnable[0Off|1On]/1(In1)  "<SensorEnable[0Off|1On]>"
  Bus Selector3/3 -> InputDataSamplePulse[0|1]/1(In1)  "<Pulse[0|1]>"
  SensorSelection_Data[0|1]/1(Out1) -> SensorScheduling/4  "SensorSelection_Data[0|1]"
  DelayPulse_SensorOutput[0|1]/1(Out1) -> SensorScheduling/5  "DelayPulse_SensorOutput[0|1]"
  Conflict_Flag[0|1]/1(Out1) -> SensorScheduling/6  "Conflict_Flag[0|1]"
  CycleConflict_Info[]/1(Out1) -> SensorScheduling/7  "CycleConflict_Info[]"
  Bus Selector3/2 -> SensorIdx_Selected[]/1(In1)  "<SensorIdx_Selected[]>"
  Bus Selector3/7 -> CycleConflict_Info[]/1(In1)  "<CylceConflict_Info[]>"
  Bus Selector3/8 -> IndexConflict_Info[]/1(In1)  "<IndexConflict_Info[]>"
  IndexConflict_Info[]/1(Out1) -> SensorScheduling/8  "IndexConflict_Info[]"
  SensorIdx_Selected[]/1(Out1) -> SensorScheduling/2  "SensorIdx_Selected[]"

== system ASM_Traffic_MultiCore/Environment/Sensors/UserInterface/DISP_Plant/Traffic_Sign_Sensor ==
  TrafficBus : Inport
  Angle_CoorSys_E[x;y;z][deg] : Subsystem
      mask Display: disp('')
  Angle_Hor_Rel[deg] : Subsystem
      mask Display: disp('')
  Angle_Ver_Rel[] : Subsystem
      mask Display: disp('')
  Bus Selector1 : BusSelector  OutputSignals=TrafficSign_Sensor_Dyn.Sensor_Front_1
  Bus Selector2 : BusSelector  OutputSignals=Info.TrafficSignSensor_Dyn_Sfcn_State[],Info.TrafficSignSensor_Dyn_Data_Valid[0|1]
  Distance[m] : Subsystem
      mask Display: disp('')
  GetTrfSgnDataByIndex_1 : Subsystem
  Object_State[] : Subsystem
      mask Display: disp('')
  Object_Stream_ID[] : Subsystem
      mask Display: disp('')
  Parent_Object_ID[] : Subsystem
      mask Display: disp('')
  Pos_CoorSys_E[x;y;z][m] : Subsystem
      mask Display: disp('')
  Pos_CoorSys_S[x;y;z][m] : Subsystem
      mask Display: disp('')
  Select_TrafficSign_1 : Constant
  Sign_Valid[0|1] : Subsystem
      mask Display: disp('')
  TrafficObject_ID[] : Subsystem
      mask Display: disp('')
  TrafficObject_Type[] : Subsystem
      mask Display: disp('')
  TrafficSignSensor_Data_Valid[0|1] : Subsystem
      mask Display: disp('')
  TrafficSignSensor_Sfcn_State[] : Subsystem
      mask Display: disp('')
  TrafficSign_Sensor_Dynamic_ObjectData : Scope  NumInputPorts=4
      settings: TimeSpan=5  ActiveDisplayYMinimum=0  ActiveDisplayYMaximum=1  DataLoggingMaxPoints=20000  DataLoggingDecimation=10  DataLoggingVariableName=ScopeData32
  TrafficSign_Sensor_Dynamic_ObjectPosition : Scope  NumInputPorts=6
      settings: TimeSpan=5  ActiveDisplayYMinimum=0  ActiveDisplayYMaximum=1  DataLoggingMaxPoints=20000  DataLoggingDecimation=10
  TrafficSign_Sensor_Dynamic_ObjectPosition1 : Scope  NumInputPorts=8
      settings: TimeSpan=5  ActiveDisplayYMinimum=0  ActiveDisplayYMaximum=1  DataLoggingMaxPoints=20000  DataLoggingDecimation=10  DataLoggingVariableName=ScopeData2
  TrafficSign_Sensor_Info : Scope  NumInputPorts=2
      settings: TimeSpan=5  ActiveDisplayYMinimum=0  ActiveDisplayYMaximum=1  DataLoggingMaxPoints=20000  DataLoggingDecimation=10  DataLoggingVariableName=ScopeData24
  Traffic_Sign_Country[] : Subsystem
      mask Display: disp('')
  Traffic_Sign_Lanes[] : Subsystem
      mask Display: disp('')
  Traffic_Sign_Subtype[] : Subsystem
      mask Display: disp('')
  Traffic_Sign_Type[] : Subsystem
      mask Display: disp('')
  Traffic_Sign_Value[] : Subsystem
      mask Display: disp('')
  Traffic_Sign_Visibility[0_100] : Subsystem
      mask Display: disp('')
  wires:
  Traffic_Sign_Lanes[]/1(Out1) -> TrafficSign_Sensor_Dynamic_ObjectPosition1/8  "Traffic_Sign_Lanes[]"
  Object_Stream_ID[]/1(Out1) -> TrafficSign_Sensor_Dynamic_ObjectPosition1/7  "Object_Stream_ID[]"
  Object_State[]/1(Out1) -> TrafficSign_Sensor_Dynamic_ObjectPosition1/6  "Object_State[]"
  GetTrfSgnDataByIndex_1/18(Traffic_Sign_Lanes[]) -> Traffic_Sign_Lanes[]/1(In1)
  GetTrfSgnDataByIndex_1/17(Object_Stream_ID[]) -> Object_Stream_ID[]/1(In1)
  GetTrfSgnDataByIndex_1/16(Object_State[]) -> Object_State[]/1(In1)
  Traffic_Sign_Country[]/1(Out1) -> TrafficSign_Sensor_Dynamic_ObjectPosition1/4  "Traffic_Sign_Country[]"
  GetTrfSgnDataByIndex_1/15(Traffic_Sign_Visibility[0_100]) -> Traffic_Sign_Visibility[0_100]/1(In1)
  Traffic_Sign_Subtype[]/1(Out1) -> TrafficSign_Sensor_Dynamic_ObjectPosition1/2  "Traffic_Sign_Subtype[]"
  Traffic_Sign_Type[]/1(Out1) -> TrafficSign_Sensor_Dynamic_ObjectPosition1/1  "Traffic_Sign_Type[]"
  GetTrfSgnDataByIndex_1/14(Traffic_Sign_Country[]) -> Traffic_Sign_Country[]/1(In1)
  GetTrfSgnDataByIndex_1/13(Traffic_Sign_Value[]) -> Traffic_Sign_Value[]/1(In1)
  GetTrfSgnDataByIndex_1/12(Traffic_Sign_Subtype[]) -> Traffic_Sign_Subtype[]/1(In1)
  GetTrfSgnDataByIndex_1/11(Traffic_Sign_Type[]) -> Traffic_Sign_Type[]/1(In1)
  Distance[m]/1(Out1) -> TrafficSign_Sensor_Dynamic_ObjectPosition/6  "Distance[m]"
  Angle_Ver_Rel[]/1(Out1) -> TrafficSign_Sensor_Dynamic_ObjectPosition/5  "Angle_Ver_Rel[]"
  Angle_Hor_Rel[deg]/1(Out1) -> TrafficSign_Sensor_Dynamic_ObjectPosition/4  "Angle_Hor_Rel[deg]"
  Pos_CoorSys_S[x;y;z][m]/1(Out1) -> TrafficSign_Sensor_Dynamic_ObjectPosition/3  "Pos_CoorSys_S[x;y;z][m]"
  Angle_CoorSys_E[x;y;z][deg]/1(Out1) -> TrafficSign_Sensor_Dynamic_ObjectPosition/2  "Angle_CoorSys_E[x;y;z][deg]"
  Pos_CoorSys_E[x;y;z][m]/1(Out1) -> TrafficSign_Sensor_Dynamic_ObjectPosition/1  "Pos_CoorSys_E[x;y;z][m]"
  GetTrfSgnDataByIndex_1/10(Distance[m]) -> Distance[m]/1(In1)
  GetTrfSgnDataByIndex_1/9(Angle_Ver_Rel[deg]) -> Angle_Ver_Rel[]/1(In1)
  GetTrfSgnDataByIndex_1/8(Angle_Hor_Rel[deg]) -> Angle_Hor_Rel[deg]/1(In1)
  GetTrfSgnDataByIndex_1/7(Pos_CoorSys_S[x;y;z][m]) -> Pos_CoorSys_S[x;y;z][m]/1(In1)
  GetTrfSgnDataByIndex_1/6(Angle_CoorSys_E[x;y;z][deg]) -> Angle_CoorSys_E[x;y;z][deg]/1(In1)
  GetTrfSgnDataByIndex_1/5(Pos_CoorSys_E[x;y;z][m]) -> Pos_CoorSys_E[x;y;z][m]/1(In1)
  Parent_Object_ID[]/1(Out1) -> TrafficSign_Sensor_Dynamic_ObjectData/4  "Parent_Object_ID[]"
  TrafficObject_Type[]/1(Out1) -> TrafficSign_Sensor_Dynamic_ObjectData/3  "TrafficObject_Type[]"
  Sign_Valid[0|1]/1(Out1) -> TrafficSign_Sensor_Dynamic_ObjectData/1  "Sign_Valid[0|1]"
  TrafficObject_ID[]/1(Out1) -> TrafficSign_Sensor_Dynamic_ObjectData/2  "TrafficObject_ID[]"
  GetTrfSgnDataByIndex_1/4(Parent_Object_ID[]) -> Parent_Object_ID[]/1(In1)
  GetTrfSgnDataByIndex_1/3(TrafficObject_Type[]) -> TrafficObject_Type[]/1(In1)
  GetTrfSgnDataByIndex_1/2(TrafficObject_ID[]) -> TrafficObject_ID[]/1(In1)
  GetTrfSgnDataByIndex_1/1(Traffic_Sign_Valid[0|1]) -> Sign_Valid[0|1]/1(In1)
  Select_TrafficSign_1/1 -> GetTrfSgnDataByIndex_1/1(SelectSignDataByIndex)
  Traffic_Sign_Visibility[0_100]/1(Out1) -> TrafficSign_Sensor_Dynamic_ObjectPosition1/5  "Traffic_Sign_Visibility[0_100]"
  Traffic_Sign_Value[]/1(Out1) -> TrafficSign_Sensor_Dynamic_ObjectPosition1/3  "Traffic_Sign_Value[]"
  TrafficSignSensor_Sfcn_State[]/1(Out1) -> TrafficSign_Sensor_Info/1  "TrafficSignSensor_Sfcn_State[]"
  TrafficSignSensor_Data_Valid[0|1]/1(Out1) -> TrafficSign_Sensor_Info/2  "TrafficSignSensor_Data_Valid[0|1]"
  Bus Selector2/2 -> TrafficSignSensor_Data_Valid[0|1]/1(In1)  "<TrafficSignSensor_Dyn_Data_Valid[0|1]>"
  Bus Selector2/1 -> TrafficSignSensor_Sfcn_State[]/1(In1)  "<TrafficSignSensor_Dyn_Sfcn_State[]>"
  TrafficBus/1 -> Bus Selector1/1, GetTrfSgnDataByIndex_1/2(TrafficBus)
  Bus Selector1/1 -> Bus Selector2/1  "<Sensor_Front_1>"

== system ASM_Traffic_MultiCore/Environment/SignalInterface/ASMSignalInterface/signal_structure/InfoBlock ==

== system ASM_Traffic_MultiCore/Environment/Traffic/PlantModel/FellowMovement/ASMSignalBusCollect ==
  d_Total_Fellows_Road[m] : Inport
  LaneIdx_Total_Fellows_Road[] : Inport  Port=2
  s_Fellows_Road[m] : Inport  Port=3
  v_Fellows_In[km|h] : Inport  Port=4
  Bus Creator2 : BusCreator  Inputs=4
  avoid_incomplete_trace2source : Subsystem
  avoid_incomplete_trace2source1 : Subsystem
  avoid_incomplete_trace2source2 : Subsystem
  avoid_incomplete_trace2source3 : Subsystem
  ASMSignalBus : Outport  VectorParamsAs1DForOutWhenUnconnected=off
  wires:
  avoid_incomplete_trace2source3/1(Out1) -> Bus Creator2/4  "v_Fellows[km|h]"
  avoid_incomplete_trace2source2/1(Out1) -> Bus Creator2/3  "s_Fellows[m]"
  avoid_incomplete_trace2source1/1(Out1) -> Bus Creator2/2  "LaneIdx_Total_Fellows[]"
  avoid_incomplete_trace2source/1(Out1) -> Bus Creator2/1  "d_Total_Fellows[m]"
  d_Total_Fellows_Road[m]/1 -> avoid_incomplete_trace2source/1(In1)
  LaneIdx_Total_Fellows_Road[]/1 -> avoid_incomplete_trace2source1/1(In1)
  s_Fellows_Road[m]/1 -> avoid_incomplete_trace2source2/1(In1)
  v_Fellows_In[km|h]/1 -> avoid_incomplete_trace2source3/1(In1)
  Bus Creator2/1 -> ASMSignalBus/1  "FellowSignalLabels"

== system ASM_Traffic_MultiCore/Environment/Traffic/PlantModel/FellowMovement/ASMSignalCollector ==
  FellowPosVel : Inport
  Bus Creator1 : BusCreator  Inputs=5
  Bus Selector : BusSelector  OutputSignals=FellowPositions,FellowVelocities
  FellowMovement_Signals : Outport  VectorParamsAs1DForOutWhenUnconnected=off
  wires:
  Bus Selector/2 -> Bus Creator1/3  "<FellowVelocities>"
  Bus Selector/1 -> Bus Creator1/2  "<FellowPositions>"
  FellowPosVel/1 -> Bus Selector/1
  [ASMBUS_Traffic_UserSignals_Customized] -> Bus Creator1/5
  [ASMBUS_Traffic_TrafficScheduler] -> Bus Creator1/4
  [ASMBUS_Traffic_FellowSignalLabels] -> Bus Creator1/1
  Bus Creator1/1 -> FellowMovement_Signals/1  "FellowMovement"
